simulink model "FDIR_SensorFault_Subsystem"  (R2026a)
settings: Solver=FixedStepDiscrete  StopTime=0.1  FixedStep=0.01
settings Model: Creator=ekanshsingh  LastModifiedBy=ekanshsingh

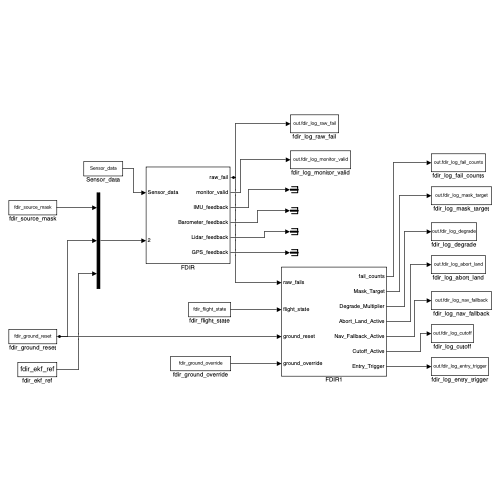
[thumbnail: Simulink's stored preview of the top-level diagram]
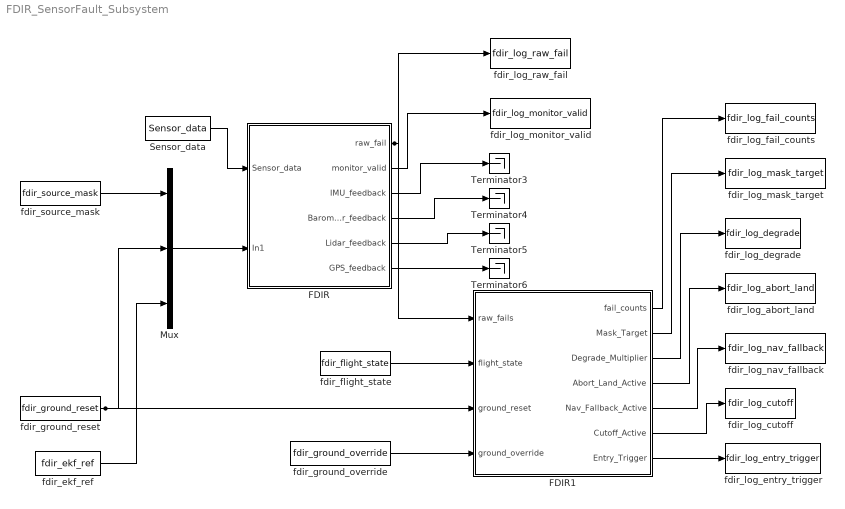
== system FDIR_SensorFault_Subsystem ==
  FDIR : Subsystem
  FDIR1 : Subsystem
  Mux : Mux  Inputs=3
  Sensor_data : FromWorkspace  VariableName=Sensor_data  SampleTime=0.01  OutputAfterFinalValue=Holding final value
  Terminator{3..6} (4 alike) : Terminator
  fdir_ekf_ref : FromWorkspace  VariableName=fdir_ekf_ref  SampleTime=0.01  OutputAfterFinalValue=Holding final value
  fdir_flight_state : FromWorkspace  VariableName=fdir_flight_state  SampleTime=0.01  OutputAfterFinalValue=Holding final value
  fdir_ground_override : FromWorkspace  VariableName=fdir_ground_override  SampleTime=0.01  OutputAfterFinalValue=Holding final value
  fdir_ground_reset : FromWorkspace  VariableName=fdir_ground_reset  SampleTime=0.01  OutputAfterFinalValue=Holding final value
  fdir_log_abort_land : ToWorkspace  VariableName=fdir_log_abort_land  SaveFormat=Timeseries  SampleTime=-1
  fdir_log_cutoff : ToWorkspace  VariableName=fdir_log_cutoff  SaveFormat=Timeseries  SampleTime=-1
  fdir_log_degrade : ToWorkspace  VariableName=fdir_log_degrade  SaveFormat=Timeseries  SampleTime=-1
  fdir_log_entry_trigger : ToWorkspace  VariableName=fdir_log_entry_trigger  SaveFormat=Timeseries  SampleTime=-1
  fdir_log_fail_counts : ToWorkspace  VariableName=fdir_log_fail_counts  SaveFormat=Timeseries  SampleTime=-1
  fdir_log_mask_target : ToWorkspace  VariableName=fdir_log_mask_target  SaveFormat=Timeseries  SampleTime=-1
  fdir_log_monitor_valid : ToWorkspace  VariableName=fdir_log_monitor_valid  SaveFormat=Timeseries  SampleTime=-1
  fdir_log_nav_fallback : ToWorkspace  VariableName=fdir_log_nav_fallback  SaveFormat=Timeseries  SampleTime=-1
  fdir_log_raw_fail : ToWorkspace  VariableName=fdir_log_raw_fail  SaveFormat=Timeseries  SampleTime=-1
  fdir_source_mask : FromWorkspace  VariableName=fdir_source_mask  SampleTime=0.01  OutputAfterFinalValue=Holding final value
  wires:
  FDIR1/6(Cutoff_Active) -> fdir_log_cutoff/1
  FDIR1/5(Nav_Fallback_Active) -> fdir_log_nav_fallback/1
  FDIR1/4(Abort_Land_Active) -> fdir_log_abort_land/1
  FDIR1/3(Degrade_Multiplier) -> fdir_log_degrade/1
  FDIR1/1(fail_counts) -> fdir_log_fail_counts/1
  fdir_ground_override/1 -> FDIR1/4(ground_override)
  Sensor_data/1 -> FDIR/1(Sensor_data)
  FDIR/2(monitor_valid) -> fdir_log_monitor_valid/1
  FDIR/1(raw_fail) -> fdir_log_raw_fail/1, FDIR1/1(raw_fails)
  FDIR/3(IMU_feedback) -> Terminator3/1
  Mux/1 -> FDIR/2(In1)
  FDIR/6(GPS_feedback) -> Terminator6/1
  FDIR1/2(Mask_Target) -> fdir_log_mask_target/1
  fdir_ekf_ref/1 -> Mux/3
  FDIR/4(Barometer_feedback) -> Terminator4/1
  FDIR1/7(Entry_Trigger) -> fdir_log_entry_trigger/1
  fdir_ground_reset/1 -> Mux/2, FDIR1/3(ground_reset)
  fdir_flight_state/1 -> FDIR1/2(flight_state)
  FDIR/5(Lidar_feedback) -> Terminator5/1
  fdir_source_mask/1 -> Mux/1

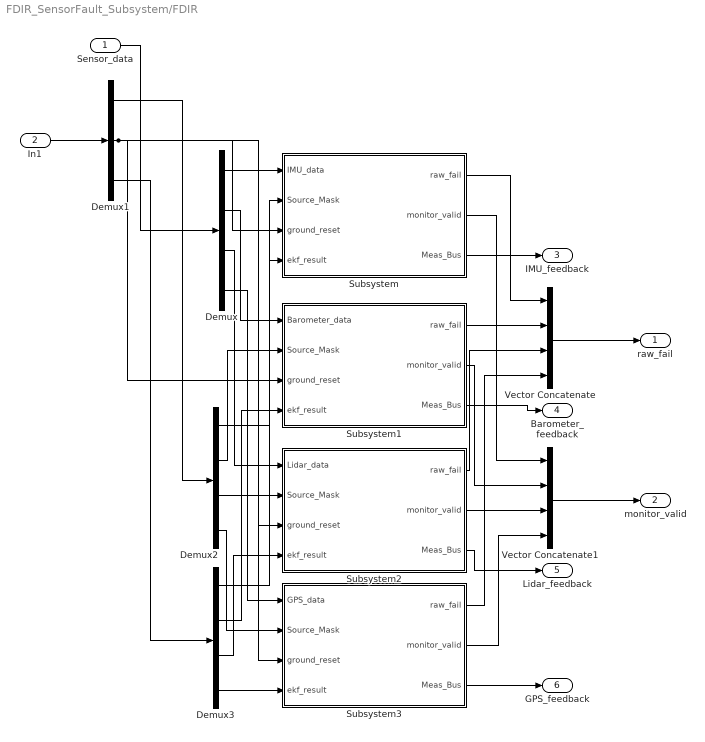
== system FDIR_SensorFault_Subsystem/FDIR ==
  Sensor_data : Inport
  In1 : Inport  Port=2
  Demux : Demux  Outputs=[6 1 1 3]
  Demux1 : Demux  Outputs=[4 1 11]
  Demux2 : Demux
  Demux3 : Demux  Outputs=[6 1 1 3]
  Subsystem : Subsystem
  Subsystem1 : Subsystem
  Subsystem2 : Subsystem
  Subsystem3 : Subsystem
  Vector Concatenate : Concatenate  NumInputs=4
  Vector Concatenate1 : Concatenate  NumInputs=4
  raw_fail : Outport
  monitor_valid : Outport  Port=2
  IMU_feedback : Outport  Port=3
  Barometer_feedback : Outport  Port=4
  Lidar_feedback : Outport  Port=5
  GPS_feedback : Outport  Port=6
  wires:
  Vector Concatenate1/1 -> monitor_valid/1
  Subsystem3/3(Meas_Bus) -> GPS_feedback/1
  Subsystem3/2(monitor_valid) -> Vector Concatenate1/4
  Subsystem2/3(Meas_Bus) -> Lidar_feedback/1
  Subsystem1/3(Meas_Bus) -> Barometer_feedback/1
  Subsystem1/2(monitor_valid) -> Vector Concatenate1/2
  Subsystem/3(Meas_Bus) -> IMU_feedback/1
  Demux3/4 -> Subsystem3/4(ekf_result)
  Demux3/3 -> Subsystem2/4(ekf_result)
  Demux3/2 -> Subsystem1/4(ekf_result)
  Demux3/1 -> Subsystem/4(ekf_result)
  Subsystem/2(monitor_valid) -> Vector Concatenate1/1
  Demux2/4 -> Subsystem3/2(Source_Mask)
  Demux2/3 -> Subsystem2/2(Source_Mask)
  Demux/3 -> Subsystem2/1(Lidar_data)
  Sensor_data/1 -> Demux/1
  Subsystem2/1(raw_fail) -> Vector Concatenate/3
  Demux2/2 -> Subsystem1/2(Source_Mask)
  Demux1/1 -> Demux2/1
  Subsystem/1(raw_fail) -> Vector Concatenate/1
  Subsystem2/2(monitor_valid) -> Vector Concatenate1/3
  Demux/2 -> Subsystem1/1(Barometer_data)
  Subsystem3/1(raw_fail) -> Vector Concatenate/4
  Demux1/3 -> Demux3/1
  Demux2/1 -> Subsystem/2(Source_Mask)
  Demux/1 -> Subsystem/1(IMU_data)
  Demux1/2 -> Subsystem/3(ground_reset), Subsystem3/3(ground_reset), Subsystem1/3(ground_reset), Subsystem2/3(ground_reset)
  Vector Concatenate/1 -> raw_fail/1
  Demux/4 -> Subsystem3/1(GPS_data)
  Subsystem1/1(raw_fail) -> Vector Concatenate/2
  In1/1 -> Demux1/1

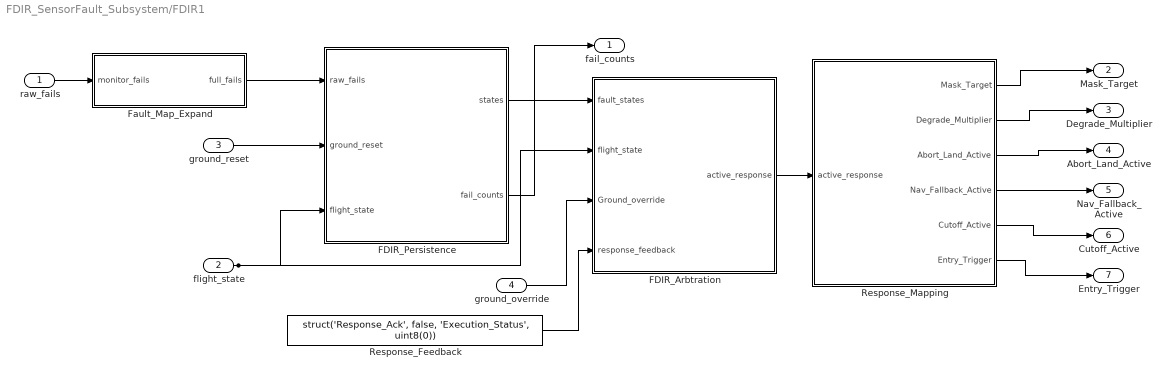
== system FDIR_SensorFault_Subsystem/FDIR1 ==
  raw_fails : Inport
  flight_state : Inport  Port=2
  ground_reset : Inport  Port=3
  ground_override : Inport  Port=4
  FDIR_Arbtration : MATLAB Function  TreatAsAtomicUnit=on
  FDIR_Persistence : MATLAB Function  TreatAsAtomicUnit=on
  Fault_Map_Expand : MATLAB Function  TreatAsAtomicUnit=on
  Response_Feedback : Constant  Value=struct('Response_Ack', false, 'Execution_Status', uint8(0))  OutDataTypeStr=Bus: Response_Feedback_Bus
  Response_Mapping : MATLAB Function  TreatAsAtomicUnit=on
  fail_counts : Outport
  Mask_Target : Outport  Port=2
  Degrade_Multiplier : Outport  Port=3
  Abort_Land_Active : Outport  Port=4
  Nav_Fallback_Active : Outport  Port=5
  Cutoff_Active : Outport  Port=6
  Entry_Trigger : Outport  Port=7
  wires:
  Response_Mapping/5(Cutoff_Active) -> Cutoff_Active/1
  Response_Mapping/4(Nav_Fallback_Active) -> Nav_Fallback_Active/1
  Response_Mapping/1(Mask_Target) -> Mask_Target/1
  FDIR_Arbtration/1(active_response) -> Response_Mapping/1(active_response)
  ground_override/1 -> FDIR_Arbtration/3(Ground_override)
  Response_Mapping/6(Entry_Trigger) -> Entry_Trigger/1
  FDIR_Persistence/2(fail_counts) -> fail_counts/1
  Response_Mapping/3(Abort_Land_Active) -> Abort_Land_Active/1
  Fault_Map_Expand/1(full_fails) -> FDIR_Persistence/1(raw_fails)
  flight_state/1 -> FDIR_Persistence/3(flight_state), FDIR_Arbtration/2(flight_state)
  FDIR_Persistence/1(states) -> FDIR_Arbtration/1(fault_states)
  raw_fails/1 -> Fault_Map_Expand/1(monitor_fails)
  ground_reset/1 -> FDIR_Persistence/2(ground_reset)
  Response_Mapping/2(Degrade_Multiplier) -> Degrade_Multiplier/1
  Response_Feedback/1 -> FDIR_Arbtration/4(response_feedback)

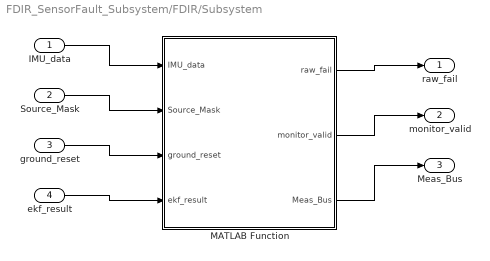
== system FDIR_SensorFault_Subsystem/FDIR/Subsystem ==
  IMU_data : Inport
  Source_Mask : Inport  Port=2
  ground_reset : Inport  Port=3
  ekf_result : Inport  Port=4
  MATLAB Function : MATLAB Function  TreatAsAtomicUnit=on
  raw_fail : Outport
  monitor_valid : Outport  Port=2
  Meas_Bus : Outport  Port=3
  wires:
  IMU_data/1 -> MATLAB Function/1(IMU_data)
  Source_Mask/1 -> MATLAB Function/2(Source_Mask)
  ground_reset/1 -> MATLAB Function/3(ground_reset)
  ekf_result/1 -> MATLAB Function/4(ekf_result)
  MATLAB Function/1(raw_fail) -> raw_fail/1
  MATLAB Function/2(monitor_valid) -> monitor_valid/1
  MATLAB Function/3(Meas_Bus) -> Meas_Bus/1

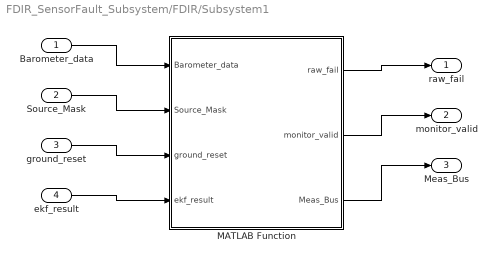
== system FDIR_SensorFault_Subsystem/FDIR/Subsystem1 ==
  Barometer_data : Inport
  Source_Mask : Inport  Port=2
  ground_reset : Inport  Port=3
  ekf_result : Inport  Port=4
  MATLAB Function : MATLAB Function  TreatAsAtomicUnit=on
  raw_fail : Outport
  monitor_valid : Outport  Port=2
  Meas_Bus : Outport  Port=3
  wires:
  Barometer_data/1 -> MATLAB Function/1(Barometer_data)
  Source_Mask/1 -> MATLAB Function/2(Source_Mask)
  ground_reset/1 -> MATLAB Function/3(ground_reset)
  ekf_result/1 -> MATLAB Function/4(ekf_result)
  MATLAB Function/1(raw_fail) -> raw_fail/1
  MATLAB Function/2(monitor_valid) -> monitor_valid/1
  MATLAB Function/3(Meas_Bus) -> Meas_Bus/1

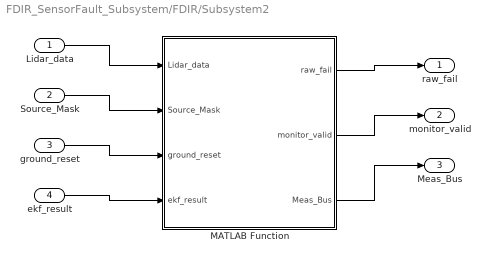
== system FDIR_SensorFault_Subsystem/FDIR/Subsystem2 ==
  Lidar_data : Inport
  Source_Mask : Inport  Port=2
  ground_reset : Inport  Port=3
  ekf_result : Inport  Port=4
  MATLAB Function : MATLAB Function  TreatAsAtomicUnit=on
  raw_fail : Outport
  monitor_valid : Outport  Port=2
  Meas_Bus : Outport  Port=3
  wires:
  Lidar_data/1 -> MATLAB Function/1(Lidar_data)
  Source_Mask/1 -> MATLAB Function/2(Source_Mask)
  ground_reset/1 -> MATLAB Function/3(ground_reset)
  ekf_result/1 -> MATLAB Function/4(ekf_result)
  MATLAB Function/1(raw_fail) -> raw_fail/1
  MATLAB Function/2(monitor_valid) -> monitor_valid/1
  MATLAB Function/3(Meas_Bus) -> Meas_Bus/1

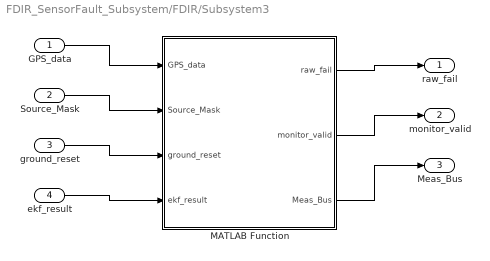
== system FDIR_SensorFault_Subsystem/FDIR/Subsystem3 ==
  GPS_data : Inport
  Source_Mask : Inport  Port=2
  ground_reset : Inport  Port=3
  ekf_result : Inport  Port=4
  MATLAB Function : MATLAB Function  TreatAsAtomicUnit=on
  raw_fail : Outport
  monitor_valid : Outport  Port=2
  Meas_Bus : Outport  Port=3
  wires:
  GPS_data/1 -> MATLAB Function/1(GPS_data)
  Source_Mask/1 -> MATLAB Function/2(Source_Mask)
  ground_reset/1 -> MATLAB Function/3(ground_reset)
  ekf_result/1 -> MATLAB Function/4(ekf_result)
  MATLAB Function/1(raw_fail) -> raw_fail/1
  MATLAB Function/2(monitor_valid) -> monitor_valid/1
  MATLAB Function/3(Meas_Bus) -> Meas_Bus/1

== matlab function FDIR_SensorFault_Subsystem/FDIR/Subsystem1/MATLAB Function ==
  data: Barometer_data input; raw_fail output; Source_Mask input; ground_reset input; ekf_result input; monitor_valid output; Meas_Bus output
function [raw_fail, monitor_valid, Meas_Bus] = fcn(Barometer_data, Source_Mask, ground_reset, ekf_result)
%#codegen
% Thin wrapper - the logic lives in fdir_sensor_monitor.m.
persistent mon_state
if isempty(mon_state)
    mon_state = fdir_monitor_state(1);
end
C = fdir_config();
[raw_fail, monitor_valid, Meas_Bus, mon_state] = fdir_sensor_monitor( ...
    Barometer_data, ekf_result, Source_Mask, ground_reset, C.sensors.Barometer, mon_state);
end

== matlab function FDIR_SensorFault_Subsystem/FDIR/Subsystem/MATLAB Function ==
  data: IMU_data input; raw_fail output; Source_Mask input; ground_reset input; ekf_result input; monitor_valid output; Meas_Bus output
function [raw_fail, monitor_valid, Meas_Bus] = fcn(IMU_data, Source_Mask, ground_reset, ekf_result)
%#codegen
% Thin wrapper - the logic lives in fdir_sensor_monitor.m.
persistent mon_state
if isempty(mon_state)
    mon_state = fdir_monitor_state(6);
end
C = fdir_config();
[raw_fail, monitor_valid, Meas_Bus, mon_state] = fdir_sensor_monitor( ...
    IMU_data, ekf_result, Source_Mask, ground_reset, C.sensors.IMU, mon_state);
end

== matlab function FDIR_SensorFault_Subsystem/FDIR/Subsystem2/MATLAB Function ==
  data: Lidar_data input; raw_fail output; Source_Mask input; ground_reset input; ekf_result input; monitor_valid output; Meas_Bus output
function [raw_fail, monitor_valid, Meas_Bus] = fcn(Lidar_data, Source_Mask, ground_reset, ekf_result)
%#codegen
% Thin wrapper - the logic lives in fdir_sensor_monitor.m.
persistent mon_state
if isempty(mon_state)
    mon_state = fdir_monitor_state(1);
end
C = fdir_config();
[raw_fail, monitor_valid, Meas_Bus, mon_state] = fdir_sensor_monitor( ...
    Lidar_data, ekf_result, Source_Mask, ground_reset, C.sensors.Lidar, mon_state);
end

== matlab function FDIR_SensorFault_Subsystem/FDIR/Subsystem3/MATLAB Function ==
  data: GPS_data input; raw_fail output; Source_Mask input; ground_reset input; ekf_result input; monitor_valid output; Meas_Bus output
function [raw_fail, monitor_valid, Meas_Bus] = fcn(GPS_data, Source_Mask, ground_reset, ekf_result)
%#codegen
% Thin wrapper - the logic lives in fdir_sensor_monitor.m.
persistent mon_state
if isempty(mon_state)
    mon_state = fdir_monitor_state(3);
end
C = fdir_config();
[raw_fail, monitor_valid, Meas_Bus, mon_state] = fdir_sensor_monitor( ...
    GPS_data, ekf_result, Source_Mask, ground_reset, C.sensors.GPS, mon_state);
end

== matlab function FDIR_SensorFault_Subsystem/FDIR1/Fault_Map_Expand ==
  data: monitor_fails input; full_fails output
function full_fails = fcn(monitor_fails)
%#codegen
% Thin wrapper - the logic lives in fdir_expand_raw_fails.m.
% 16 monitor checks -> 102 catalog-indexed faults.
C = fdir_config();
full_fails = fdir_expand_raw_fails(monitor_fails, C.fault_map, 102);
end

== matlab function FDIR_SensorFault_Subsystem/FDIR1/FDIR_Persistence ==
  data: raw_fails input; states output Bus: Fault_State_Bus size=102; ground_reset input; flight_state input; fail_counts output
function [states, fail_counts] = fcn(raw_fails, ground_reset, flight_state)
%#codegen
% Thin wrapper - the logic lives in fdir_persistence.m.
persistent p_state
[C, fault_config] = fdir_config();
if isempty(p_state)
    p_state = fdir_persistence_state(102, C.M_WINDOW_SIZE);
end
% The ground reset command is a single discrete, applied to every fault.
ground_resets = repmat(logical(ground_reset), 102, 1);
[states, fail_counts, p_state] = fdir_persistence( ...
    raw_fails, ground_resets, flight_state, fault_config, p_state);
end

== matlab function FDIR_SensorFault_Subsystem/FDIR1/FDIR_Arbtration ==
  data: fault_states input Bus: Fault_State_Bus size=102; active_response output; flight_state input; Ground_override input; response_feedback input Bus: Response_Feedback_Bus
function active_response = fcn(fault_states, flight_state, Ground_override, response_feedback)
%#codegen
% Thin wrapper - the logic lives in fdir_arbitration.m.
persistent current_response
if isempty(current_response)
    current_response = uint8(0); % R0 (Nominal)
end
[~, fault_config] = fdir_config();
[active_response, current_response] = fdir_arbitration( ...
    fault_states, flight_state, Ground_override, response_feedback, ...
    fault_config, current_response);
end

== matlab function FDIR_SensorFault_Subsystem/FDIR1/Response_Mapping ==
  data: active_response input; Mask_Target output; Degrade_Multiplier output; Abort_Land_Active output; Nav_Fallback_Active output; Cutoff_Active output; Entry_Trigger output
function [Mask_Target, Degrade_Multiplier, Abort_Land_Active, Nav_Fallback_Active, Cutoff_Active, Entry_Trigger] = fcn(active_response)
%#codegen
% Thin wrapper - the logic lives in fdir_response_mapping.m.
[Mask_Target, Degrade_Multiplier, Abort_Land_Active, Nav_Fallback_Active, Cutoff_Active, Entry_Trigger] = ...
    fdir_response_mapping(active_response);
end
